simulink model "sschdlexViennaRectifierModel"  (R2026a)
settings: Solver=FixedStepDiscrete  StopTime=0.8  MaxStep=1e-4
PreLoadFcn:
  | % Copyright 2017-2023 The MathWorks, Inc.
  | 
  | %% System Parameters
  | Vs    = 120*sqrt(3); % AC source line-to-line (V, rms)
  | Vpeak = Vs/sqrt(3)*sqrt(2); % AC source line-to-ground (V, peak)
  | R = 0.1;  % Resistance (Ohm)
  | L = 2e-3; % Inductance (H)
  | Vdcnom = 400;  % Nominal output dc voltage (V)
  | Pnom   = 10e3; % Nominal power (W)
  | Imax   = Pnom/(1.5*Vpeak); % Maximum ac current        (A)
  | Inom   = Pnom/Vdcnom;      % Nominal output dc current (A)
  | Iload  = 0.2*Inom;         % Initial load current      (A)
  | 
  | %% Control Parameters
  | fsw = 5e3;        % Switching frequency (Hz)
  | Ts  = 1/(50*fsw); % Fundamental sample time (s)
  | Tsc = 1/(10*fsw); % Control sample time (s)
  | 
  | Kp_vdc = 0.7386; % Proportional gain dc-link voltage controller
  | Ki_vdc = 135.6;  % Integral gain dc-link voltage controller
  | Kp_id  = 8.407;  % Proportional gain d-axis current controller
  | Ki_id  = 1127;   % Integral gain d-axis current controller
  | Kp_iq  = 11.91;  % Proportional gain q-axis current controller
  | Ki_iq  = 3706;   % Integral gain q-axis current controller
  | Kp_vn  = 0.4912; % Proportional gain neutral voltage controller
libraries: ee_lib x27, nesl_utility x13, fl_lib x10, eeTransforms x4, slpidlib x4, eeGeneralControl x4, eePwmGeneratorViennaRectifier x1, eeSinusoidalMeasurement x1, eePowerMeasurement x1
(part 2 of 2)

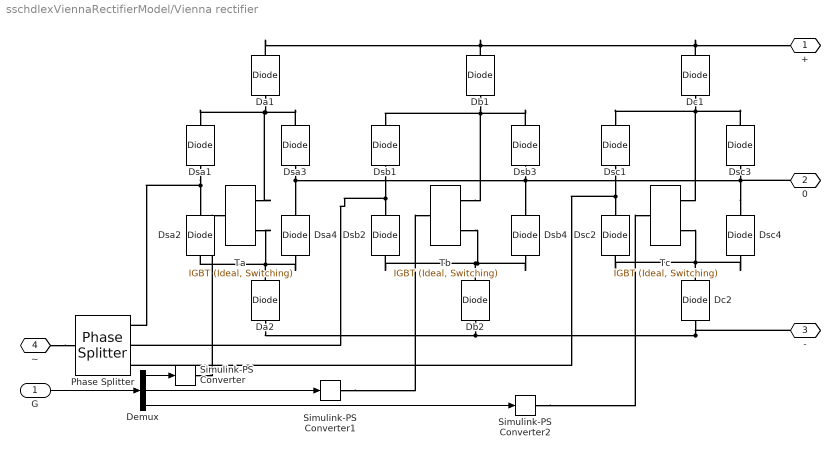
== system sschdlexViennaRectifierModel/Vienna rectifier ==
  G : Inport
  Da1 : ee_lib/Semiconductors & Converters/Diode  ModelType=ee.enum.diode.modelType.pwl  TableType=ee.enum.diode.tableType.IfMat  IfMat=[.07, .12, .19, 1.75, 4.24, 7.32, 11.2; .16, .3, .72, 2.14, 4.02, 6.35, 9.12] A  VfMat=[.9, 1.15, 1.25, 1.5, 1.75, 2.17, 2.6, 2.85; .58, .68, .75, 1.1, 1.38, 1.77, 2.27, 2.7] V  TjVec=[25, 125] degC  VfVec=[.5, .7, .9, 1.3, 1.7, 2.1, 2.5] V  IfVec=[.1, .2, .5, 1, 2, 4, 7, 10] A  IrMat=[1e-06, 2e-06, 5e-06, 1e-05, 2.5e-05, 5e-05, .0001; 2e-06, 5e-06, 1e-05, 4e-05, 8e-05, .0002, .0005] A  VrMat=[10, 100, 200, 250, 300, 325, 350; 10, 70, 160, 220, 270, 300, 320] V  VrVec=[10, 20, 40, 50, 70, 80, 100] V  IrVec=[1e-06, 2e-06, 5e-06, 1e-05, 2e-05, 5e-05, .0001] A  Vf=0.8 V  Ron=0.001 Ohm  Goff=1e-5 1/Ohm  prmExp=ee.enum.diode.expParam.useTwo  I12=[.0137, .545] A  V12=[.6, .7] V  RS=0 Ohm  Tmeas=25 degC  IS=1e-12 A  ec=1  I1=0.0137 A  V1=0.6 V  N_series=1  N_parallel=1  ZenerEnable=false  Rz=0.3 Ohm  BV=inf V  C_param=ee.enum.diode.capParam.fixed  CJ=0 pF  CJ0=5 pF  Vvec=[.1, 10, 100] V  Cvec=[3.5, 1, .4] pF  VJ=1 V  Mgrad=0.5  FC=0.5  Q_param=ee.enum.diode.recoveryParam.off  iRM=-7.15 A  iF=4 A  didt=-750 A/us  trr_factor=3  trr=115 ns  Qrr=1500 s*uA  Vr=-600 V  Ls=150 nH  Erec=0.03 J  TT=50 ns  tau=100 ns  T_param=ee.enum.diode.temperatureParam.off  Tdevice=25 degC  I1_T2=0.245 A  V1_T2=0.5 V  IS_T2=1.25e-7 A  Tmeas2=125 degC  XTI_param=ee.enum.diode.xtiParam.pn  XTI=3  EG_param=ee.enum.diode.egapParam.material_si  EG=1.11 eV  dBVdT=0 V/K  enable_fault_input=simscape.enum.onoff.off  i_specify=off  i_priority=None  i=0 A  i_nominal_specify=off  i_nominal_value=1  i_nominal_unit=A  v_specify=off  v_priority=None  v=0 V  v_nominal_specify=off  v_nominal_value=1  v_nominal_unit=V  v_capacitor_specify=off  v_capacitor_priority=None  v_capacitor=0 V  v_capacitor_nominal_specify=off  v_capacitor_nominal_value=1  v_capacitor_nominal_unit=V  Qj_specify=off  Qj_priority=High  Qj=0 C  Qj_nominal_specify=off  Qj_nominal_value=1  Qj_nominal_unit=C  i_diode_specify=off  i_diode_priority=None  i_diode=0 A  i_diode_nominal_specify=off  i_diode_nominal_value=1  i_diode_nominal_unit=A  v_diode_specify=off  v_diode_priority=None  v_diode=0 V  v_diode_nominal_specify=off  v_diode_nominal_value=1  v_diode_nominal_unit=V  i_capacitor_specify=off  i_capacitor_priority=None  i_capacitor=0 A  i_capacitor_nominal_specify=off  i_capacitor_nominal_value=1  i_capacitor_nominal_unit=A  fidelity_level=ee.enum.diode.fidelity.includeChargeDyn  rec_loss_model=ee.enum.diode.reverseRecoveryModel.fixed  ErecVal=0 J  scaleWithIandV=true  ErecMat=zeros(2, 3) J  ErecMat3D=zeros(2, 3, 2) J  TjrecVec=[298.15, 398.15] K  IfrecVec=[.1, 1, 10] A  IrecVal=10 A  VrecVal=10 V  VrecVec=[0, 100] V  tFilter=1 / 1000 / 100 s  thermal_network_parameterization=ee.enum.thermalNetworkTopology.junctionCase  Rth=[0, 10] K/W  Rth_Cauer=[1, 3, 10] K/W  Rth_Foster=[4, 6] K/W  thermal_mass_parameterization=ee.enum.thermalNetwork.timeconstant  thermal_mass=[0, 1] J/K  thermal_mass_Cauer=[.1, .3, 1] J/K  thermal_mass_Foster=[1.5, 3] J/K  thermal_time_constant=[0, 10] s  thermal_time_constant_Cauer=[1, 3, 10] s  thermal_time_constant_Foster=[6, 18] s  thermal_mass_initial_temperatures=[25, 25] degC  thermal_mass_initial_temperatures_Cauer=[25, 25, 25] degC  junction_thermal_mass=0.01 J/K  Tvec_initial_Foster=[25, 25, 25, 25] degC  no_thermal_network=0  junction_temperature_specify=off  junction_temperature_priority=None  junction_temperature=25 degC  junction_temperature_nominal_specify=off  junction_temperature_nominal_value=1  junction_temperature_nominal_unit=degC
  Da2 : ee_lib/Semiconductors & Converters/Diode  ModelType=ee.enum.diode.modelType.pwl  TableType=ee.enum.diode.tableType.IfMat  IfMat=[.07, .12, .19, 1.75, 4.24, 7.32, 11.2; .16, .3, .72, 2.14, 4.02, 6.35, 9.12] A  VfMat=[.9, 1.15, 1.25, 1.5, 1.75, 2.17, 2.6, 2.85; .58, .68, .75, 1.1, 1.38, 1.77, 2.27, 2.7] V  TjVec=[25, 125] degC  VfVec=[.5, .7, .9, 1.3, 1.7, 2.1, 2.5] V  IfVec=[.1, .2, .5, 1, 2, 4, 7, 10] A  IrMat=[1e-06, 2e-06, 5e-06, 1e-05, 2.5e-05, 5e-05, .0001; 2e-06, 5e-06, 1e-05, 4e-05, 8e-05, .0002, .0005] A  VrMat=[10, 100, 200, 250, 300, 325, 350; 10, 70, 160, 220, 270, 300, 320] V  VrVec=[10, 20, 40, 50, 70, 80, 100] V  IrVec=[1e-06, 2e-06, 5e-06, 1e-05, 2e-05, 5e-05, .0001] A  Vf=0.8 V  Ron=0.001 Ohm  Goff=1e-5 1/Ohm  prmExp=ee.enum.diode.expParam.useTwo  I12=[.0137, .545] A  V12=[.6, .7] V  RS=0 Ohm  Tmeas=25 degC  IS=1e-12 A  ec=1  I1=0.0137 A  V1=0.6 V  N_series=1  N_parallel=1  ZenerEnable=false  Rz=0.3 Ohm  BV=inf V  C_param=ee.enum.diode.capParam.fixed  CJ=0 pF  CJ0=5 pF  Vvec=[.1, 10, 100] V  Cvec=[3.5, 1, .4] pF  VJ=1 V  Mgrad=0.5  FC=0.5  Q_param=ee.enum.diode.recoveryParam.off  iRM=-7.15 A  iF=4 A  didt=-750 A/us  trr_factor=3  trr=115 ns  Qrr=1500 s*uA  Vr=-600 V  Ls=150 nH  Erec=0.03 J  TT=50 ns  tau=100 ns  T_param=ee.enum.diode.temperatureParam.off  Tdevice=25 degC  I1_T2=0.245 A  V1_T2=0.5 V  IS_T2=1.25e-7 A  Tmeas2=125 degC  XTI_param=ee.enum.diode.xtiParam.pn  XTI=3  EG_param=ee.enum.diode.egapParam.material_si  EG=1.11 eV  dBVdT=0 V/K  enable_fault_input=simscape.enum.onoff.off  i_specify=off  i_priority=None  i=0 A  i_nominal_specify=off  i_nominal_value=1  i_nominal_unit=A  v_specify=off  v_priority=None  v=0 V  v_nominal_specify=off  v_nominal_value=1  v_nominal_unit=V  v_capacitor_specify=off  v_capacitor_priority=None  v_capacitor=0 V  v_capacitor_nominal_specify=off  v_capacitor_nominal_value=1  v_capacitor_nominal_unit=V  Qj_specify=off  Qj_priority=High  Qj=0 C  Qj_nominal_specify=off  Qj_nominal_value=1  Qj_nominal_unit=C  i_diode_specify=off  i_diode_priority=None  i_diode=0 A  i_diode_nominal_specify=off  i_diode_nominal_value=1  i_diode_nominal_unit=A  v_diode_specify=off  v_diode_priority=None  v_diode=0 V  v_diode_nominal_specify=off  v_diode_nominal_value=1  v_diode_nominal_unit=V  i_capacitor_specify=off  i_capacitor_priority=None  i_capacitor=0 A  i_capacitor_nominal_specify=off  i_capacitor_nominal_value=1  i_capacitor_nominal_unit=A  fidelity_level=ee.enum.diode.fidelity.includeChargeDyn  rec_loss_model=ee.enum.diode.reverseRecoveryModel.fixed  ErecVal=0 J  scaleWithIandV=true  ErecMat=zeros(2, 3) J  ErecMat3D=zeros(2, 3, 2) J  TjrecVec=[298.15, 398.15] K  IfrecVec=[.1, 1, 10] A  IrecVal=10 A  VrecVal=10 V  VrecVec=[0, 100] V  tFilter=1 / 1000 / 100 s  thermal_network_parameterization=ee.enum.thermalNetworkTopology.junctionCase  Rth=[0, 10] K/W  Rth_Cauer=[1, 3, 10] K/W  Rth_Foster=[4, 6] K/W  thermal_mass_parameterization=ee.enum.thermalNetwork.timeconstant  thermal_mass=[0, 1] J/K  thermal_mass_Cauer=[.1, .3, 1] J/K  thermal_mass_Foster=[1.5, 3] J/K  thermal_time_constant=[0, 10] s  thermal_time_constant_Cauer=[1, 3, 10] s  thermal_time_constant_Foster=[6, 18] s  thermal_mass_initial_temperatures=[25, 25] degC  thermal_mass_initial_temperatures_Cauer=[25, 25, 25] degC  junction_thermal_mass=0.01 J/K  Tvec_initial_Foster=[25, 25, 25, 25] degC  no_thermal_network=0  junction_temperature_specify=off  junction_temperature_priority=None  junction_temperature=25 degC  junction_temperature_nominal_specify=off  junction_temperature_nominal_value=1  junction_temperature_nominal_unit=degC
  Db1 : ee_lib/Semiconductors & Converters/Diode  ModelType=ee.enum.diode.modelType.pwl  TableType=ee.enum.diode.tableType.IfMat  IfMat=[.07, .12, .19, 1.75, 4.24, 7.32, 11.2; .16, .3, .72, 2.14, 4.02, 6.35, 9.12] A  VfMat=[.9, 1.15, 1.25, 1.5, 1.75, 2.17, 2.6, 2.85; .58, .68, .75, 1.1, 1.38, 1.77, 2.27, 2.7] V  TjVec=[25, 125] degC  VfVec=[.5, .7, .9, 1.3, 1.7, 2.1, 2.5] V  IfVec=[.1, .2, .5, 1, 2, 4, 7, 10] A  IrMat=[1e-06, 2e-06, 5e-06, 1e-05, 2.5e-05, 5e-05, .0001; 2e-06, 5e-06, 1e-05, 4e-05, 8e-05, .0002, .0005] A  VrMat=[10, 100, 200, 250, 300, 325, 350; 10, 70, 160, 220, 270, 300, 320] V  VrVec=[10, 20, 40, 50, 70, 80, 100] V  IrVec=[1e-06, 2e-06, 5e-06, 1e-05, 2e-05, 5e-05, .0001] A  Vf=0.8 V  Ron=0.001 Ohm  Goff=1e-5 1/Ohm  prmExp=ee.enum.diode.expParam.useTwo  I12=[.0137, .545] A  V12=[.6, .7] V  RS=0 Ohm  Tmeas=25 degC  IS=1e-12 A  ec=1  I1=0.0137 A  V1=0.6 V  N_series=1  N_parallel=1  ZenerEnable=false  Rz=0.3 Ohm  BV=inf V  C_param=ee.enum.diode.capParam.fixed  CJ=0 pF  CJ0=5 pF  Vvec=[.1, 10, 100] V  Cvec=[3.5, 1, .4] pF  VJ=1 V  Mgrad=0.5  FC=0.5  Q_param=ee.enum.diode.recoveryParam.off  iRM=-7.15 A  iF=4 A  didt=-750 A/us  trr_factor=3  trr=115 ns  Qrr=1500 s*uA  Vr=-600 V  Ls=150 nH  Erec=0.03 J  TT=50 ns  tau=100 ns  T_param=ee.enum.diode.temperatureParam.off  Tdevice=25 degC  I1_T2=0.245 A  V1_T2=0.5 V  IS_T2=1.25e-7 A  Tmeas2=125 degC  XTI_param=ee.enum.diode.xtiParam.pn  XTI=3  EG_param=ee.enum.diode.egapParam.material_si  EG=1.11 eV  dBVdT=0 V/K  enable_fault_input=simscape.enum.onoff.off  i_specify=off  i_priority=None  i=0 A  i_nominal_specify=off  i_nominal_value=1  i_nominal_unit=A  v_specify=off  v_priority=None  v=0 V  v_nominal_specify=off  v_nominal_value=1  v_nominal_unit=V  v_capacitor_specify=off  v_capacitor_priority=None  v_capacitor=0 V  v_capacitor_nominal_specify=off  v_capacitor_nominal_value=1  v_capacitor_nominal_unit=V  Qj_specify=off  Qj_priority=High  Qj=0 C  Qj_nominal_specify=off  Qj_nominal_value=1  Qj_nominal_unit=C  i_diode_specify=off  i_diode_priority=None  i_diode=0 A  i_diode_nominal_specify=off  i_diode_nominal_value=1  i_diode_nominal_unit=A  v_diode_specify=off  v_diode_priority=None  v_diode=0 V  v_diode_nominal_specify=off  v_diode_nominal_value=1  v_diode_nominal_unit=V  i_capacitor_specify=off  i_capacitor_priority=None  i_capacitor=0 A  i_capacitor_nominal_specify=off  i_capacitor_nominal_value=1  i_capacitor_nominal_unit=A  fidelity_level=ee.enum.diode.fidelity.includeChargeDyn  rec_loss_model=ee.enum.diode.reverseRecoveryModel.fixed  ErecVal=0 J  scaleWithIandV=true  ErecMat=zeros(2, 3) J  ErecMat3D=zeros(2, 3, 2) J  TjrecVec=[298.15, 398.15] K  IfrecVec=[.1, 1, 10] A  IrecVal=10 A  VrecVal=10 V  VrecVec=[0, 100] V  tFilter=1 / 1000 / 100 s  thermal_network_parameterization=ee.enum.thermalNetworkTopology.junctionCase  Rth=[0, 10] K/W  Rth_Cauer=[1, 3, 10] K/W  Rth_Foster=[4, 6] K/W  thermal_mass_parameterization=ee.enum.thermalNetwork.timeconstant  thermal_mass=[0, 1] J/K  thermal_mass_Cauer=[.1, .3, 1] J/K  thermal_mass_Foster=[1.5, 3] J/K  thermal_time_constant=[0, 10] s  thermal_time_constant_Cauer=[1, 3, 10] s  thermal_time_constant_Foster=[6, 18] s  thermal_mass_initial_temperatures=[25, 25] degC  thermal_mass_initial_temperatures_Cauer=[25, 25, 25] degC  junction_thermal_mass=0.01 J/K  Tvec_initial_Foster=[25, 25, 25, 25] degC  no_thermal_network=0  junction_temperature_specify=off  junction_temperature_priority=None  junction_temperature=25 degC  junction_temperature_nominal_specify=off  junction_temperature_nominal_value=1  junction_temperature_nominal_unit=degC
  Db2 : ee_lib/Semiconductors & Converters/Diode  ModelType=ee.enum.diode.modelType.pwl  TableType=ee.enum.diode.tableType.IfMat  IfMat=[.07, .12, .19, 1.75, 4.24, 7.32, 11.2; .16, .3, .72, 2.14, 4.02, 6.35, 9.12] A  VfMat=[.9, 1.15, 1.25, 1.5, 1.75, 2.17, 2.6, 2.85; .58, .68, .75, 1.1, 1.38, 1.77, 2.27, 2.7] V  TjVec=[25, 125] degC  VfVec=[.5, .7, .9, 1.3, 1.7, 2.1, 2.5] V  IfVec=[.1, .2, .5, 1, 2, 4, 7, 10] A  IrMat=[1e-06, 2e-06, 5e-06, 1e-05, 2.5e-05, 5e-05, .0001; 2e-06, 5e-06, 1e-05, 4e-05, 8e-05, .0002, .0005] A  VrMat=[10, 100, 200, 250, 300, 325, 350; 10, 70, 160, 220, 270, 300, 320] V  VrVec=[10, 20, 40, 50, 70, 80, 100] V  IrVec=[1e-06, 2e-06, 5e-06, 1e-05, 2e-05, 5e-05, .0001] A  Vf=0.8 V  Ron=0.001 Ohm  Goff=1e-5 1/Ohm  prmExp=ee.enum.diode.expParam.useTwo  I12=[.0137, .545] A  V12=[.6, .7] V  RS=0 Ohm  Tmeas=25 degC  IS=1e-12 A  ec=1  I1=0.0137 A  V1=0.6 V  N_series=1  N_parallel=1  ZenerEnable=false  Rz=0.3 Ohm  BV=inf V  C_param=ee.enum.diode.capParam.fixed  CJ=0 pF  CJ0=5 pF  Vvec=[.1, 10, 100] V  Cvec=[3.5, 1, .4] pF  VJ=1 V  Mgrad=0.5  FC=0.5  Q_param=ee.enum.diode.recoveryParam.off  iRM=-7.15 A  iF=4 A  didt=-750 A/us  trr_factor=3  trr=115 ns  Qrr=1500 s*uA  Vr=-600 V  Ls=150 nH  Erec=0.03 J  TT=50 ns  tau=100 ns  T_param=ee.enum.diode.temperatureParam.off  Tdevice=25 degC  I1_T2=0.245 A  V1_T2=0.5 V  IS_T2=1.25e-7 A  Tmeas2=125 degC  XTI_param=ee.enum.diode.xtiParam.pn  XTI=3  EG_param=ee.enum.diode.egapParam.material_si  EG=1.11 eV  dBVdT=0 V/K  enable_fault_input=simscape.enum.onoff.off  i_specify=off  i_priority=None  i=0 A  i_nominal_specify=off  i_nominal_value=1  i_nominal_unit=A  v_specify=off  v_priority=None  v=0 V  v_nominal_specify=off  v_nominal_value=1  v_nominal_unit=V  v_capacitor_specify=off  v_capacitor_priority=None  v_capacitor=0 V  v_capacitor_nominal_specify=off  v_capacitor_nominal_value=1  v_capacitor_nominal_unit=V  Qj_specify=off  Qj_priority=High  Qj=0 C  Qj_nominal_specify=off  Qj_nominal_value=1  Qj_nominal_unit=C  i_diode_specify=off  i_diode_priority=None  i_diode=0 A  i_diode_nominal_specify=off  i_diode_nominal_value=1  i_diode_nominal_unit=A  v_diode_specify=off  v_diode_priority=None  v_diode=0 V  v_diode_nominal_specify=off  v_diode_nominal_value=1  v_diode_nominal_unit=V  i_capacitor_specify=off  i_capacitor_priority=None  i_capacitor=0 A  i_capacitor_nominal_specify=off  i_capacitor_nominal_value=1  i_capacitor_nominal_unit=A  fidelity_level=ee.enum.diode.fidelity.includeChargeDyn  rec_loss_model=ee.enum.diode.reverseRecoveryModel.fixed  ErecVal=0 J  scaleWithIandV=true  ErecMat=zeros(2, 3) J  ErecMat3D=zeros(2, 3, 2) J  TjrecVec=[298.15, 398.15] K  IfrecVec=[.1, 1, 10] A  IrecVal=10 A  VrecVal=10 V  VrecVec=[0, 100] V  tFilter=1 / 1000 / 100 s  thermal_network_parameterization=ee.enum.thermalNetworkTopology.junctionCase  Rth=[0, 10] K/W  Rth_Cauer=[1, 3, 10] K/W  Rth_Foster=[4, 6] K/W  thermal_mass_parameterization=ee.enum.thermalNetwork.timeconstant  thermal_mass=[0, 1] J/K  thermal_mass_Cauer=[.1, .3, 1] J/K  thermal_mass_Foster=[1.5, 3] J/K  thermal_time_constant=[0, 10] s  thermal_time_constant_Cauer=[1, 3, 10] s  thermal_time_constant_Foster=[6, 18] s  thermal_mass_initial_temperatures=[25, 25] degC  thermal_mass_initial_temperatures_Cauer=[25, 25, 25] degC  junction_thermal_mass=0.01 J/K  Tvec_initial_Foster=[25, 25, 25, 25] degC  no_thermal_network=0  junction_temperature_specify=off  junction_temperature_priority=None  junction_temperature=25 degC  junction_temperature_nominal_specify=off  junction_temperature_nominal_value=1  junction_temperature_nominal_unit=degC
  Dc1 : ee_lib/Semiconductors & Converters/Diode  ModelType=ee.enum.diode.modelType.pwl  TableType=ee.enum.diode.tableType.IfMat  IfMat=[.07, .12, .19, 1.75, 4.24, 7.32, 11.2; .16, .3, .72, 2.14, 4.02, 6.35, 9.12] A  VfMat=[.9, 1.15, 1.25, 1.5, 1.75, 2.17, 2.6, 2.85; .58, .68, .75, 1.1, 1.38, 1.77, 2.27, 2.7] V  TjVec=[25, 125] degC  VfVec=[.5, .7, .9, 1.3, 1.7, 2.1, 2.5] V  IfVec=[.1, .2, .5, 1, 2, 4, 7, 10] A  IrMat=[1e-06, 2e-06, 5e-06, 1e-05, 2.5e-05, 5e-05, .0001; 2e-06, 5e-06, 1e-05, 4e-05, 8e-05, .0002, .0005] A  VrMat=[10, 100, 200, 250, 300, 325, 350; 10, 70, 160, 220, 270, 300, 320] V  VrVec=[10, 20, 40, 50, 70, 80, 100] V  IrVec=[1e-06, 2e-06, 5e-06, 1e-05, 2e-05, 5e-05, .0001] A  Vf=0.8 V  Ron=0.001 Ohm  Goff=1e-5 1/Ohm  prmExp=ee.enum.diode.expParam.useTwo  I12=[.0137, .545] A  V12=[.6, .7] V  RS=0 Ohm  Tmeas=25 degC  IS=1e-12 A  ec=1  I1=0.0137 A  V1=0.6 V  N_series=1  N_parallel=1  ZenerEnable=false  Rz=0.3 Ohm  BV=inf V  C_param=ee.enum.diode.capParam.fixed  CJ=0 pF  CJ0=5 pF  Vvec=[.1, 10, 100] V  Cvec=[3.5, 1, .4] pF  VJ=1 V  Mgrad=0.5  FC=0.5  Q_param=ee.enum.diode.recoveryParam.off  iRM=-7.15 A  iF=4 A  didt=-750 A/us  trr_factor=3  trr=115 ns  Qrr=1500 s*uA  Vr=-600 V  Ls=150 nH  Erec=0.03 J  TT=50 ns  tau=100 ns  T_param=ee.enum.diode.temperatureParam.off  Tdevice=25 degC  I1_T2=0.245 A  V1_T2=0.5 V  IS_T2=1.25e-7 A  Tmeas2=125 degC  XTI_param=ee.enum.diode.xtiParam.pn  XTI=3  EG_param=ee.enum.diode.egapParam.material_si  EG=1.11 eV  dBVdT=0 V/K  enable_fault_input=simscape.enum.onoff.off  i_specify=off  i_priority=None  i=0 A  i_nominal_specify=off  i_nominal_value=1  i_nominal_unit=A  v_specify=off  v_priority=None  v=0 V  v_nominal_specify=off  v_nominal_value=1  v_nominal_unit=V  v_capacitor_specify=off  v_capacitor_priority=None  v_capacitor=0 V  v_capacitor_nominal_specify=off  v_capacitor_nominal_value=1  v_capacitor_nominal_unit=V  Qj_specify=off  Qj_priority=High  Qj=0 C  Qj_nominal_specify=off  Qj_nominal_value=1  Qj_nominal_unit=C  i_diode_specify=off  i_diode_priority=None  i_diode=0 A  i_diode_nominal_specify=off  i_diode_nominal_value=1  i_diode_nominal_unit=A  v_diode_specify=off  v_diode_priority=None  v_diode=0 V  v_diode_nominal_specify=off  v_diode_nominal_value=1  v_diode_nominal_unit=V  i_capacitor_specify=off  i_capacitor_priority=None  i_capacitor=0 A  i_capacitor_nominal_specify=off  i_capacitor_nominal_value=1  i_capacitor_nominal_unit=A  fidelity_level=ee.enum.diode.fidelity.includeChargeDyn  rec_loss_model=ee.enum.diode.reverseRecoveryModel.fixed  ErecVal=0 J  scaleWithIandV=true  ErecMat=zeros(2, 3) J  ErecMat3D=zeros(2, 3, 2) J  TjrecVec=[298.15, 398.15] K  IfrecVec=[.1, 1, 10] A  IrecVal=10 A  VrecVal=10 V  VrecVec=[0, 100] V  tFilter=1 / 1000 / 100 s  thermal_network_parameterization=ee.enum.thermalNetworkTopology.junctionCase  Rth=[0, 10] K/W  Rth_Cauer=[1, 3, 10] K/W  Rth_Foster=[4, 6] K/W  thermal_mass_parameterization=ee.enum.thermalNetwork.timeconstant  thermal_mass=[0, 1] J/K  thermal_mass_Cauer=[.1, .3, 1] J/K  thermal_mass_Foster=[1.5, 3] J/K  thermal_time_constant=[0, 10] s  thermal_time_constant_Cauer=[1, 3, 10] s  thermal_time_constant_Foster=[6, 18] s  thermal_mass_initial_temperatures=[25, 25] degC  thermal_mass_initial_temperatures_Cauer=[25, 25, 25] degC  junction_thermal_mass=0.01 J/K  Tvec_initial_Foster=[25, 25, 25, 25] degC  no_thermal_network=0  junction_temperature_specify=off  junction_temperature_priority=None  junction_temperature=25 degC  junction_temperature_nominal_specify=off  junction_temperature_nominal_value=1  junction_temperature_nominal_unit=degC
  Dc2 : ee_lib/Semiconductors & Converters/Diode  ModelType=ee.enum.diode.modelType.pwl  TableType=ee.enum.diode.tableType.IfMat  IfMat=[.07, .12, .19, 1.75, 4.24, 7.32, 11.2; .16, .3, .72, 2.14, 4.02, 6.35, 9.12] A  VfMat=[.9, 1.15, 1.25, 1.5, 1.75, 2.17, 2.6, 2.85; .58, .68, .75, 1.1, 1.38, 1.77, 2.27, 2.7] V  TjVec=[25, 125] degC  VfVec=[.5, .7, .9, 1.3, 1.7, 2.1, 2.5] V  IfVec=[.1, .2, .5, 1, 2, 4, 7, 10] A  IrMat=[1e-06, 2e-06, 5e-06, 1e-05, 2.5e-05, 5e-05, .0001; 2e-06, 5e-06, 1e-05, 4e-05, 8e-05, .0002, .0005] A  VrMat=[10, 100, 200, 250, 300, 325, 350; 10, 70, 160, 220, 270, 300, 320] V  VrVec=[10, 20, 40, 50, 70, 80, 100] V  IrVec=[1e-06, 2e-06, 5e-06, 1e-05, 2e-05, 5e-05, .0001] A  Vf=0.8 V  Ron=0.001 Ohm  Goff=1e-5 1/Ohm  prmExp=ee.enum.diode.expParam.useTwo  I12=[.0137, .545] A  V12=[.6, .7] V  RS=0 Ohm  Tmeas=25 degC  IS=1e-12 A  ec=1  I1=0.0137 A  V1=0.6 V  N_series=1  N_parallel=1  ZenerEnable=false  Rz=0.3 Ohm  BV=inf V  C_param=ee.enum.diode.capParam.fixed  CJ=0 pF  CJ0=5 pF  Vvec=[.1, 10, 100] V  Cvec=[3.5, 1, .4] pF  VJ=1 V  Mgrad=0.5  FC=0.5  Q_param=ee.enum.diode.recoveryParam.off  iRM=-7.15 A  iF=4 A  didt=-750 A/us  trr_factor=3  trr=115 ns  Qrr=1500 s*uA  Vr=-600 V  Ls=150 nH  Erec=0.03 J  TT=50 ns  tau=100 ns  T_param=ee.enum.diode.temperatureParam.off  Tdevice=25 degC  I1_T2=0.245 A  V1_T2=0.5 V  IS_T2=1.25e-7 A  Tmeas2=125 degC  XTI_param=ee.enum.diode.xtiParam.pn  XTI=3  EG_param=ee.enum.diode.egapParam.material_si  EG=1.11 eV  dBVdT=0 V/K  enable_fault_input=simscape.enum.onoff.off  i_specify=off  i_priority=None  i=0 A  i_nominal_specify=off  i_nominal_value=1  i_nominal_unit=A  v_specify=off  v_priority=None  v=0 V  v_nominal_specify=off  v_nominal_value=1  v_nominal_unit=V  v_capacitor_specify=off  v_capacitor_priority=None  v_capacitor=0 V  v_capacitor_nominal_specify=off  v_capacitor_nominal_value=1  v_capacitor_nominal_unit=V  Qj_specify=off  Qj_priority=High  Qj=0 C  Qj_nominal_specify=off  Qj_nominal_value=1  Qj_nominal_unit=C  i_diode_specify=off  i_diode_priority=None  i_diode=0 A  i_diode_nominal_specify=off  i_diode_nominal_value=1  i_diode_nominal_unit=A  v_diode_specify=off  v_diode_priority=None  v_diode=0 V  v_diode_nominal_specify=off  v_diode_nominal_value=1  v_diode_nominal_unit=V  i_capacitor_specify=off  i_capacitor_priority=None  i_capacitor=0 A  i_capacitor_nominal_specify=off  i_capacitor_nominal_value=1  i_capacitor_nominal_unit=A  fidelity_level=ee.enum.diode.fidelity.includeChargeDyn  rec_loss_model=ee.enum.diode.reverseRecoveryModel.fixed  ErecVal=0 J  scaleWithIandV=true  ErecMat=zeros(2, 3) J  ErecMat3D=zeros(2, 3, 2) J  TjrecVec=[298.15, 398.15] K  IfrecVec=[.1, 1, 10] A  IrecVal=10 A  VrecVal=10 V  VrecVec=[0, 100] V  tFilter=1 / 1000 / 100 s  thermal_network_parameterization=ee.enum.thermalNetworkTopology.junctionCase  Rth=[0, 10] K/W  Rth_Cauer=[1, 3, 10] K/W  Rth_Foster=[4, 6] K/W  thermal_mass_parameterization=ee.enum.thermalNetwork.timeconstant  thermal_mass=[0, 1] J/K  thermal_mass_Cauer=[.1, .3, 1] J/K  thermal_mass_Foster=[1.5, 3] J/K  thermal_time_constant=[0, 10] s  thermal_time_constant_Cauer=[1, 3, 10] s  thermal_time_constant_Foster=[6, 18] s  thermal_mass_initial_temperatures=[25, 25] degC  thermal_mass_initial_temperatures_Cauer=[25, 25, 25] degC  junction_thermal_mass=0.01 J/K  Tvec_initial_Foster=[25, 25, 25, 25] degC  no_thermal_network=0  junction_temperature_specify=off  junction_temperature_priority=None  junction_temperature=25 degC  junction_temperature_nominal_specify=off  junction_temperature_nominal_value=1  junction_temperature_nominal_unit=degC
  Demux : Demux  Outputs=3
  Dsa{1..4} (4 alike) : ee_lib/Semiconductors & Converters/Diode  ModelType=ee.enum.diode.modelType.pwl  TableType=ee.enum.diode.tableType.IfMat  IfMat=[.07, .12, .19, 1.75, 4.24, 7.32, 11.2; .16, .3, .72, 2.14, 4.02, 6.35, 9.12] A  VfMat=[.9, 1.15, 1.25, 1.5, 1.75, 2.17, 2.6, 2.85; .58, .68, .75, 1.1, 1.38, 1.77, 2.27, 2.7] V  TjVec=[25, 125] degC  VfVec=[.5, .7, .9, 1.3, 1.7, 2.1, 2.5] V  IfVec=[.1, .2, .5, 1, 2, 4, 7, 10] A  IrMat=[1e-06, 2e-06, 5e-06, 1e-05, 2.5e-05, 5e-05, .0001; 2e-06, 5e-06, 1e-05, 4e-05, 8e-05, .0002, .0005] A  VrMat=[10, 100, 200, 250, 300, 325, 350; 10, 70, 160, 220, 270, 300, 320] V  VrVec=[10, 20, 40, 50, 70, 80, 100] V  IrVec=[1e-06, 2e-06, 5e-06, 1e-05, 2e-05, 5e-05, .0001] A  Vf=0.8 V  Ron=0.001 Ohm  Goff=1e-5 1/Ohm  prmExp=ee.enum.diode.expParam.useTwo  I12=[.0137, .545] A  V12=[.6, .7] V  RS=0 Ohm  Tmeas=25 degC  IS=1e-12 A  ec=1  I1=0.0137 A  V1=0.6 V  N_series=1  N_parallel=1  ZenerEnable=false  Rz=0.3 Ohm  BV=inf V  C_param=ee.enum.diode.capParam.fixed  CJ=0 pF  CJ0=5 pF  Vvec=[.1, 10, 100] V  Cvec=[3.5, 1, .4] pF  VJ=1 V  Mgrad=0.5  FC=0.5  Q_param=ee.enum.diode.recoveryParam.off  iRM=-7.15 A  iF=4 A  didt=-750 A/us  trr_factor=3  trr=115 ns  Qrr=1500 s*uA  Vr=-600 V  Ls=150 nH  Erec=0.03 J  TT=50 ns  tau=100 ns  T_param=ee.enum.diode.temperatureParam.off  Tdevice=25 degC  I1_T2=0.245 A  V1_T2=0.5 V  IS_T2=1.25e-7 A  Tmeas2=125 degC  XTI_param=ee.enum.diode.xtiParam.pn  XTI=3  EG_param=ee.enum.diode.egapParam.material_si  EG=1.11 eV  dBVdT=0 V/K  enable_fault_input=simscape.enum.onoff.off  i_specify=off  i_priority=None  i=0 A  i_nominal_specify=off  i_nominal_value=1  i_nominal_unit=A  v_specify=off  v_priority=None  v=0 V  v_nominal_specify=off  v_nominal_value=1  v_nominal_unit=V  v_capacitor_specify=off  v_capacitor_priority=None  v_capacitor=0 V  v_capacitor_nominal_specify=off  v_capacitor_nominal_value=1  v_capacitor_nominal_unit=V  Qj_specify=off  Qj_priority=High  Qj=0 C  Qj_nominal_specify=off  Qj_nominal_value=1  Qj_nominal_unit=C  i_diode_specify=off  i_diode_priority=None  i_diode=0 A  i_diode_nominal_specify=off  i_diode_nominal_value=1  i_diode_nominal_unit=A  v_diode_specify=off  v_diode_priority=None  v_diode=0 V  v_diode_nominal_specify=off  v_diode_nominal_value=1  v_diode_nominal_unit=V  i_capacitor_specify=off  i_capacitor_priority=None  i_capacitor=0 A  i_capacitor_nominal_specify=off  i_capacitor_nominal_value=1  i_capacitor_nominal_unit=A  fidelity_level=ee.enum.diode.fidelity.includeChargeDyn  rec_loss_model=ee.enum.diode.reverseRecoveryModel.fixed  ErecVal=0 J  scaleWithIandV=true  ErecMat=zeros(2, 3) J  ErecMat3D=zeros(2, 3, 2) J  TjrecVec=[298.15, 398.15] K  IfrecVec=[.1, 1, 10] A  IrecVal=10 A  VrecVal=10 V  VrecVec=[0, 100] V  tFilter=1 / 1000 / 100 s  thermal_network_parameterization=ee.enum.thermalNetworkTopology.junctionCase  Rth=[0, 10] K/W  Rth_Cauer=[1, 3, 10] K/W  Rth_Foster=[4, 6] K/W  thermal_mass_parameterization=ee.enum.thermalNetwork.timeconstant  thermal_mass=[0, 1] J/K  thermal_mass_Cauer=[.1, .3, 1] J/K  thermal_mass_Foster=[1.5, 3] J/K  thermal_time_constant=[0, 10] s  thermal_time_constant_Cauer=[1, 3, 10] s  thermal_time_constant_Foster=[6, 18] s  thermal_mass_initial_temperatures=[25, 25] degC  thermal_mass_initial_temperatures_Cauer=[25, 25, 25] degC  junction_thermal_mass=0.01 J/K  Tvec_initial_Foster=[25, 25, 25, 25] degC  no_thermal_network=0  junction_temperature_specify=off  junction_temperature_priority=None  junction_temperature=25 degC  junction_temperature_nominal_specify=off  junction_temperature_nominal_value=1  junction_temperature_nominal_unit=degC
  Dsb{1..4} (4 alike) : ee_lib/Semiconductors & Converters/Diode  ModelType=ee.enum.diode.modelType.pwl  TableType=ee.enum.diode.tableType.IfMat  IfMat=[.07, .12, .19, 1.75, 4.24, 7.32, 11.2; .16, .3, .72, 2.14, 4.02, 6.35, 9.12] A  VfMat=[.9, 1.15, 1.25, 1.5, 1.75, 2.17, 2.6, 2.85; .58, .68, .75, 1.1, 1.38, 1.77, 2.27, 2.7] V  TjVec=[25, 125] degC  VfVec=[.5, .7, .9, 1.3, 1.7, 2.1, 2.5] V  IfVec=[.1, .2, .5, 1, 2, 4, 7, 10] A  IrMat=[1e-06, 2e-06, 5e-06, 1e-05, 2.5e-05, 5e-05, .0001; 2e-06, 5e-06, 1e-05, 4e-05, 8e-05, .0002, .0005] A  VrMat=[10, 100, 200, 250, 300, 325, 350; 10, 70, 160, 220, 270, 300, 320] V  VrVec=[10, 20, 40, 50, 70, 80, 100] V  IrVec=[1e-06, 2e-06, 5e-06, 1e-05, 2e-05, 5e-05, .0001] A  Vf=0.8 V  Ron=0.001 Ohm  Goff=1e-5 1/Ohm  prmExp=ee.enum.diode.expParam.useTwo  I12=[.0137, .545] A  V12=[.6, .7] V  RS=0 Ohm  Tmeas=25 degC  IS=1e-12 A  ec=1  I1=0.0137 A  V1=0.6 V  N_series=1  N_parallel=1  ZenerEnable=false  Rz=0.3 Ohm  BV=inf V  C_param=ee.enum.diode.capParam.fixed  CJ=0 pF  CJ0=5 pF  Vvec=[.1, 10, 100] V  Cvec=[3.5, 1, .4] pF  VJ=1 V  Mgrad=0.5  FC=0.5  Q_param=ee.enum.diode.recoveryParam.off  iRM=-7.15 A  iF=4 A  didt=-750 A/us  trr_factor=3  trr=115 ns  Qrr=1500 s*uA  Vr=-600 V  Ls=150 nH  Erec=0.03 J  TT=50 ns  tau=100 ns  T_param=ee.enum.diode.temperatureParam.off  Tdevice=25 degC  I1_T2=0.245 A  V1_T2=0.5 V  IS_T2=1.25e-7 A  Tmeas2=125 degC  XTI_param=ee.enum.diode.xtiParam.pn  XTI=3  EG_param=ee.enum.diode.egapParam.material_si  EG=1.11 eV  dBVdT=0 V/K  enable_fault_input=simscape.enum.onoff.off  i_specify=off  i_priority=None  i=0 A  i_nominal_specify=off  i_nominal_value=1  i_nominal_unit=A  v_specify=off  v_priority=None  v=0 V  v_nominal_specify=off  v_nominal_value=1  v_nominal_unit=V  v_capacitor_specify=off  v_capacitor_priority=None  v_capacitor=0 V  v_capacitor_nominal_specify=off  v_capacitor_nominal_value=1  v_capacitor_nominal_unit=V  Qj_specify=off  Qj_priority=High  Qj=0 C  Qj_nominal_specify=off  Qj_nominal_value=1  Qj_nominal_unit=C  i_diode_specify=off  i_diode_priority=None  i_diode=0 A  i_diode_nominal_specify=off  i_diode_nominal_value=1  i_diode_nominal_unit=A  v_diode_specify=off  v_diode_priority=None  v_diode=0 V  v_diode_nominal_specify=off  v_diode_nominal_value=1  v_diode_nominal_unit=V  i_capacitor_specify=off  i_capacitor_priority=None  i_capacitor=0 A  i_capacitor_nominal_specify=off  i_capacitor_nominal_value=1  i_capacitor_nominal_unit=A  fidelity_level=ee.enum.diode.fidelity.includeChargeDyn  rec_loss_model=ee.enum.diode.reverseRecoveryModel.fixed  ErecVal=0 J  scaleWithIandV=true  ErecMat=zeros(2, 3) J  ErecMat3D=zeros(2, 3, 2) J  TjrecVec=[298.15, 398.15] K  IfrecVec=[.1, 1, 10] A  IrecVal=10 A  VrecVal=10 V  VrecVec=[0, 100] V  tFilter=1 / 1000 / 100 s  thermal_network_parameterization=ee.enum.thermalNetworkTopology.junctionCase  Rth=[0, 10] K/W  Rth_Cauer=[1, 3, 10] K/W  Rth_Foster=[4, 6] K/W  thermal_mass_parameterization=ee.enum.thermalNetwork.timeconstant  thermal_mass=[0, 1] J/K  thermal_mass_Cauer=[.1, .3, 1] J/K  thermal_mass_Foster=[1.5, 3] J/K  thermal_time_constant=[0, 10] s  thermal_time_constant_Cauer=[1, 3, 10] s  thermal_time_constant_Foster=[6, 18] s  thermal_mass_initial_temperatures=[25, 25] degC  thermal_mass_initial_temperatures_Cauer=[25, 25, 25] degC  junction_thermal_mass=0.01 J/K  Tvec_initial_Foster=[25, 25, 25, 25] degC  no_thermal_network=0  junction_temperature_specify=off  junction_temperature_priority=None  junction_temperature=25 degC  junction_temperature_nominal_specify=off  junction_temperature_nominal_value=1  junction_temperature_nominal_unit=degC
  Dsc{1..4} (4 alike) : ee_lib/Semiconductors & Converters/Diode  ModelType=ee.enum.diode.modelType.pwl  TableType=ee.enum.diode.tableType.IfMat  IfMat=[.07, .12, .19, 1.75, 4.24, 7.32, 11.2; .16, .3, .72, 2.14, 4.02, 6.35, 9.12] A  VfMat=[.9, 1.15, 1.25, 1.5, 1.75, 2.17, 2.6, 2.85; .58, .68, .75, 1.1, 1.38, 1.77, 2.27, 2.7] V  TjVec=[25, 125] degC  VfVec=[.5, .7, .9, 1.3, 1.7, 2.1, 2.5] V  IfVec=[.1, .2, .5, 1, 2, 4, 7, 10] A  IrMat=[1e-06, 2e-06, 5e-06, 1e-05, 2.5e-05, 5e-05, .0001; 2e-06, 5e-06, 1e-05, 4e-05, 8e-05, .0002, .0005] A  VrMat=[10, 100, 200, 250, 300, 325, 350; 10, 70, 160, 220, 270, 300, 320] V  VrVec=[10, 20, 40, 50, 70, 80, 100] V  IrVec=[1e-06, 2e-06, 5e-06, 1e-05, 2e-05, 5e-05, .0001] A  Vf=0.8 V  Ron=0.001 Ohm  Goff=1e-5 1/Ohm  prmExp=ee.enum.diode.expParam.useTwo  I12=[.0137, .545] A  V12=[.6, .7] V  RS=0 Ohm  Tmeas=25 degC  IS=1e-12 A  ec=1  I1=0.0137 A  V1=0.6 V  N_series=1  N_parallel=1  ZenerEnable=false  Rz=0.3 Ohm  BV=inf V  C_param=ee.enum.diode.capParam.fixed  CJ=0 pF  CJ0=5 pF  Vvec=[.1, 10, 100] V  Cvec=[3.5, 1, .4] pF  VJ=1 V  Mgrad=0.5  FC=0.5  Q_param=ee.enum.diode.recoveryParam.off  iRM=-7.15 A  iF=4 A  didt=-750 A/us  trr_factor=3  trr=115 ns  Qrr=1500 s*uA  Vr=-600 V  Ls=150 nH  Erec=0.03 J  TT=50 ns  tau=100 ns  T_param=ee.enum.diode.temperatureParam.off  Tdevice=25 degC  I1_T2=0.245 A  V1_T2=0.5 V  IS_T2=1.25e-7 A  Tmeas2=125 degC  XTI_param=ee.enum.diode.xtiParam.pn  XTI=3  EG_param=ee.enum.diode.egapParam.material_si  EG=1.11 eV  dBVdT=0 V/K  enable_fault_input=simscape.enum.onoff.off  i_specify=off  i_priority=None  i=0 A  i_nominal_specify=off  i_nominal_value=1  i_nominal_unit=A  v_specify=off  v_priority=None  v=0 V  v_nominal_specify=off  v_nominal_value=1  v_nominal_unit=V  v_capacitor_specify=off  v_capacitor_priority=None  v_capacitor=0 V  v_capacitor_nominal_specify=off  v_capacitor_nominal_value=1  v_capacitor_nominal_unit=V  Qj_specify=off  Qj_priority=High  Qj=0 C  Qj_nominal_specify=off  Qj_nominal_value=1  Qj_nominal_unit=C  i_diode_specify=off  i_diode_priority=None  i_diode=0 A  i_diode_nominal_specify=off  i_diode_nominal_value=1  i_diode_nominal_unit=A  v_diode_specify=off  v_diode_priority=None  v_diode=0 V  v_diode_nominal_specify=off  v_diode_nominal_value=1  v_diode_nominal_unit=V  i_capacitor_specify=off  i_capacitor_priority=None  i_capacitor=0 A  i_capacitor_nominal_specify=off  i_capacitor_nominal_value=1  i_capacitor_nominal_unit=A  fidelity_level=ee.enum.diode.fidelity.includeChargeDyn  rec_loss_model=ee.enum.diode.reverseRecoveryModel.fixed  ErecVal=0 J  scaleWithIandV=true  ErecMat=zeros(2, 3) J  ErecMat3D=zeros(2, 3, 2) J  TjrecVec=[298.15, 398.15] K  IfrecVec=[.1, 1, 10] A  IrecVal=10 A  VrecVal=10 V  VrecVec=[0, 100] V  tFilter=1 / 1000 / 100 s  thermal_network_parameterization=ee.enum.thermalNetworkTopology.junctionCase  Rth=[0, 10] K/W  Rth_Cauer=[1, 3, 10] K/W  Rth_Foster=[4, 6] K/W  thermal_mass_parameterization=ee.enum.thermalNetwork.timeconstant  thermal_mass=[0, 1] J/K  thermal_mass_Cauer=[.1, .3, 1] J/K  thermal_mass_Foster=[1.5, 3] J/K  thermal_time_constant=[0, 10] s  thermal_time_constant_Cauer=[1, 3, 10] s  thermal_time_constant_Foster=[6, 18] s  thermal_mass_initial_temperatures=[25, 25] degC  thermal_mass_initial_temperatures_Cauer=[25, 25, 25] degC  junction_thermal_mass=0.01 J/K  Tvec_initial_Foster=[25, 25, 25, 25] degC  no_thermal_network=0  junction_temperature_specify=off  junction_temperature_priority=None  junction_temperature=25 degC  junction_temperature_nominal_specify=off  junction_temperature_nominal_value=1  junction_temperature_nominal_unit=degC
  Phase Splitter : ee_lib/Connectors & References/Phase Splitter
  Simulink-PS Converter : nesl_utility/Simulink-PS Converter  PhysicalDomain=network_engine_domain  SubClassName=ps_input  LeftPortType=input  RightPortType=output  PseudoPeriodic=off  Frequencies=[]  NoiseDistribution=none  NoiseParameters=[]  Unit=1  AffineConversion=off  FilteringAndDerivatives=provide  SimscapeFilterOrder=1  InputFilterTimeConstant=0.001  UdotUserProvided=0
  Simulink-PS Converter1 : nesl_utility/Simulink-PS Converter  PhysicalDomain=network_engine_domain  SubClassName=ps_input  LeftPortType=input  RightPortType=output  PseudoPeriodic=off  Frequencies=[]  NoiseDistribution=none  NoiseParameters=[]  Unit=1  AffineConversion=off  FilteringAndDerivatives=provide  SimscapeFilterOrder=1  InputFilterTimeConstant=0.001  UdotUserProvided=0
  Simulink-PS Converter2 : nesl_utility/Simulink-PS Converter  PhysicalDomain=network_engine_domain  SubClassName=ps_input  LeftPortType=input  RightPortType=output  PseudoPeriodic=off  Frequencies=[]  NoiseDistribution=none  NoiseParameters=[]  Unit=1  AffineConversion=off  FilteringAndDerivatives=provide  SimscapeFilterOrder=1  InputFilterTimeConstant=0.001  UdotUserProvided=0
  Ta : ee_lib/Semiconductors & Converters/IGBT (Ideal, Switching)  port_option=ee.enum.controlport.ps  Vf=0.8 V  Ron=0.001 Ohm  Goff=1e-5 1/Ohm  Vth=0.5 V  diode_param=1  diode_Vf=0.8 V  diode_Ron=0.001 Ohm  diode_Goff=1e-5 1/Ohm  diode_C=5e-8 F  diode_iRM=-235 A  diode_iF=300 A  diode_idot=-50 A/us  diode_trr_param=1  diode_trr_factor=3  diode_trr=15 us  diode_Qrr=1.5e+3 s*uA  ice_specify=off  ice_priority=None  ice=0 A  ice_nominal_specify=off  ice_nominal_value=1  ice_nominal_unit=A  vce_specify=off  vce_priority=None  vce=0 V  vce_nominal_specify=off  vce_nominal_value=1  vce_nominal_unit=V  vge_specify=off  vge_priority=None  vge=0 V  vge_nominal_specify=off  vge_nominal_value=1  vge_nominal_unit=V  thermal_loss_option=ee.enum.converters.thermalLossOption.constantvalues  Von_data=[0, .1, .6, .8, 1, 1.3, 1.6, 2, 2.4; 0, .1, .7, 1, 1.2, 1.5, 1.9, 2.4, 2.8] V  Tj=[298.15, 398.15] K  Iout_data=[0, .1, 1, 5, 10, 20, 40, 70, 100] A  tabulateWithVce=false  Eon_data=[0, .0024, .024, .12, .2, .48, 1.04, 2.16, 3.24; 0, .003, .03, .15, .25, .6, 1.3, 2.7, 4.05] * 1e-3 J  Eoff_data=[0, .0007, .0066, .033, .066, .17, .33, .83, 1.5; 0, .001, .01, .05, .1, .25, .5, 1.2, 2.2] * 1e-3 J  Eon_data_3D=[zeros(2, 9, 3)] J  Eoff_data_3D=[zeros(2, 9, 3)] J  Tj_loss=[298.15, 398.15] K  Iout_data_loss=[0, .1, 1, 5, 10, 20, 40, 70, 100] A  Vce_loss=[0, 150, 300] V  Eon_scalar=22.86e-3 J  Eoff_scalar=17.14e-3 J  Voff=300 V  Iout_scalar=600 A  useCurrentFromPreviousCycle=false  useVoltageFromPreviousCycle=false  diodeModelType=ee.enum.converters.diodeModelType.pwl  diodeTableType=ee.enum.diode.tableType.IfMat  diode_ReverseIVType=ee.enum.diode.diodeReverseIV.constant  diode_IfMat=[.07, .12, .19, 1.75, 4.24, 7.32, 11.2; .16, .3, .72, 2.14, 4.02, 6.35, 9.12] A  diode_VfMat=[.9, 1.15, 1.25, 1.5, 1.75, 2.17, 2.6, 2.85; .58, .68, .75, 1.1, 1.38, 1.77, 2.27, 2.7] V  diode_TjVec=[25, 125] degC  diode_VfVec=[.5, .7, .9, 1.3, 1.7, 2.1, 2.5] V  diode_IfVec=[.1, .2, .5, 1, 2, 4, 7, 10] A  diode_IrMat=[1e-06, 2e-06, 5e-06, 1e-05, 2.5e-05, 5e-05, .0001; 2e-06, 5e-06, 1e-05, 4e-05, 8e-05, .0002, .0005] A  diode_VrMat=[10, 100, 200, 250, 300, 325, 350; 10, 70, 160, 220, 270, 300, 320] V  diode_VrVec=[10, 20, 40, 50, 70, 80, 100] V  diode_IrVec=[1e-06, 2e-06, 5e-06, 1e-05, 2e-05, 5e-05, .0001] A  diode_Vr=-600 V  diode_Ls=150 nH  diode_Erec=0.03 J  diode_rec_loss_model=ee.enum.diode.reverseRecoveryModel.fixed  diode_ErecVal=0 J  diode_scaleWithIandV=true  diode_ErecMat=zeros(2, 3) J  diodeErecMat3D=zeros(2, 3, 2) J  diode_TjrecVec=[298.15, 398.15] K  diode_IfrecVec=[.1, 1, 10] A  diodeVrecVec=[0, 100] V  diode_IrecVal=10 A  diode_VrecVal=10 V  diode_tFilter=1 / 1000 / 100 s  separateThermalPortForDiode=false  thermal_network_parameterization=ee.enum.thermalNetworkTopology.external  Rth=[.08, .5] K/W  Rth_Cauer=[.08, .1, .5] K/W  Rth_Foster=[.08, .14, .22, .16] K/W  thermal_mass_parameterization=ee.enum.thermalNetwork.timeconstant  thermal_mass=[.01, .5] J/K  thermal_mass_Cauer=[.01, .1, .5] J/K  thermal_mass_Foster=[.001, .005, .05, .5] J/K  thermal_time_constant=[.001, .2] s  thermal_time_constant_Cauer=[.001, .1, .2] s  thermal_time_constant_Foster=[7e-05, .0007, .01, .08] s  thermal_mass_initial_temperatures=[25, 25] degC  thermal_mass_initial_temperatures_Cauer=[25, 25, 25] degC  junction_thermal_mass=0.01 J/K  Tvec_initial_Foster=[25, 25, 25, 25] degC  RthDiode=[.03, .2] K/W  RthCauerDiode=[.03, .1, .2] K/W  RthFosterDiode=[.03, .2] K/W  thermalMassDiode=[3, 25] J/K  thermalMassCauerDiode=[3, 10, 25] J/K  thermalMassFosterDiode=[33, 50] J/K  thermalTauDiode=[.1, 5] s  thermalTauCauerDiode=[.1, 1, 5] s  thermalTauFosterDiode=[1, 10] s  thermalMassInitTempDiode=[25, 25] degC  thermalMassInitTempCauerDiode=[25, 25, 25] degC  junctionthermalMassDiode=0.1 J/K  TVecInitialFosterDiode=[25, 25, 25, 25] degC  no_thermal_network=0  IGBT_junction_temperature_specify=off  IGBT_junction_temperature_priority=None  IGBT_junction_temperature=25 degC  IGBT_junction_temperature_nominal_specify=off  IGBT_junction_temperature_nominal_value=1  IGBT_junction_temperature_nominal_unit=degC  diode_junction_temperature_specify=off  diode_junction_temperature_priority=None  diode_junction_temperature=25 degC  diode_junction_temperature_nominal_specify=off  diode_junction_temperature_nominal_value=1  diode_junction_temperature_nominal_unit=degC  Qj_specify=off  Qj_priority=None  Qj=0 W  Qj_nominal_specify=off  Qj_nominal_value=1  Qj_nominal_unit=W  accumulatedSwitchingLosses_specify=off  accumulatedSwitchingLosses_priority=None  accumulatedSwitchingLosses=0 J
  Tb : ee_lib/Semiconductors & Converters/IGBT (Ideal, Switching)  port_option=ee.enum.controlport.ps  Vf=0.8 V  Ron=0.001 Ohm  Goff=1e-5 1/Ohm  Vth=0.5 V  diode_param=1  diode_Vf=0.8 V  diode_Ron=0.001 Ohm  diode_Goff=1e-5 1/Ohm  diode_C=5e-8 F  diode_iRM=-235 A  diode_iF=300 A  diode_idot=-50 A/us  diode_trr_param=1  diode_trr_factor=3  diode_trr=15 us  diode_Qrr=1.5e+3 s*uA  ice_specify=off  ice_priority=None  ice=0 A  ice_nominal_specify=off  ice_nominal_value=1  ice_nominal_unit=A  vce_specify=off  vce_priority=None  vce=0 V  vce_nominal_specify=off  vce_nominal_value=1  vce_nominal_unit=V  vge_specify=off  vge_priority=None  vge=0 V  vge_nominal_specify=off  vge_nominal_value=1  vge_nominal_unit=V  thermal_loss_option=ee.enum.converters.thermalLossOption.constantvalues  Von_data=[0, .1, .6, .8, 1, 1.3, 1.6, 2, 2.4; 0, .1, .7, 1, 1.2, 1.5, 1.9, 2.4, 2.8] V  Tj=[298.15, 398.15] K  Iout_data=[0, .1, 1, 5, 10, 20, 40, 70, 100] A  tabulateWithVce=false  Eon_data=[0, .0024, .024, .12, .2, .48, 1.04, 2.16, 3.24; 0, .003, .03, .15, .25, .6, 1.3, 2.7, 4.05] * 1e-3 J  Eoff_data=[0, .0007, .0066, .033, .066, .17, .33, .83, 1.5; 0, .001, .01, .05, .1, .25, .5, 1.2, 2.2] * 1e-3 J  Eon_data_3D=[zeros(2, 9, 3)] J  Eoff_data_3D=[zeros(2, 9, 3)] J  Tj_loss=[298.15, 398.15] K  Iout_data_loss=[0, .1, 1, 5, 10, 20, 40, 70, 100] A  Vce_loss=[0, 150, 300] V  Eon_scalar=22.86e-3 J  Eoff_scalar=17.14e-3 J  Voff=300 V  Iout_scalar=600 A  useCurrentFromPreviousCycle=false  useVoltageFromPreviousCycle=false  diodeModelType=ee.enum.converters.diodeModelType.pwl  diodeTableType=ee.enum.diode.tableType.IfMat  diode_ReverseIVType=ee.enum.diode.diodeReverseIV.constant  diode_IfMat=[.07, .12, .19, 1.75, 4.24, 7.32, 11.2; .16, .3, .72, 2.14, 4.02, 6.35, 9.12] A  diode_VfMat=[.9, 1.15, 1.25, 1.5, 1.75, 2.17, 2.6, 2.85; .58, .68, .75, 1.1, 1.38, 1.77, 2.27, 2.7] V  diode_TjVec=[25, 125] degC  diode_VfVec=[.5, .7, .9, 1.3, 1.7, 2.1, 2.5] V  diode_IfVec=[.1, .2, .5, 1, 2, 4, 7, 10] A  diode_IrMat=[1e-06, 2e-06, 5e-06, 1e-05, 2.5e-05, 5e-05, .0001; 2e-06, 5e-06, 1e-05, 4e-05, 8e-05, .0002, .0005] A  diode_VrMat=[10, 100, 200, 250, 300, 325, 350; 10, 70, 160, 220, 270, 300, 320] V  diode_VrVec=[10, 20, 40, 50, 70, 80, 100] V  diode_IrVec=[1e-06, 2e-06, 5e-06, 1e-05, 2e-05, 5e-05, .0001] A  diode_Vr=-600 V  diode_Ls=150 nH  diode_Erec=0.03 J  diode_rec_loss_model=ee.enum.diode.reverseRecoveryModel.fixed  diode_ErecVal=0 J  diode_scaleWithIandV=true  diode_ErecMat=zeros(2, 3) J  diodeErecMat3D=zeros(2, 3, 2) J  diode_TjrecVec=[298.15, 398.15] K  diode_IfrecVec=[.1, 1, 10] A  diodeVrecVec=[0, 100] V  diode_IrecVal=10 A  diode_VrecVal=10 V  diode_tFilter=1 / 1000 / 100 s  separateThermalPortForDiode=false  thermal_network_parameterization=ee.enum.thermalNetworkTopology.external  Rth=[.08, .5] K/W  Rth_Cauer=[.08, .1, .5] K/W  Rth_Foster=[.08, .14, .22, .16] K/W  thermal_mass_parameterization=ee.enum.thermalNetwork.timeconstant  thermal_mass=[.01, .5] J/K  thermal_mass_Cauer=[.01, .1, .5] J/K  thermal_mass_Foster=[.001, .005, .05, .5] J/K  thermal_time_constant=[.001, .2] s  thermal_time_constant_Cauer=[.001, .1, .2] s  thermal_time_constant_Foster=[7e-05, .0007, .01, .08] s  thermal_mass_initial_temperatures=[25, 25] degC  thermal_mass_initial_temperatures_Cauer=[25, 25, 25] degC  junction_thermal_mass=0.01 J/K  Tvec_initial_Foster=[25, 25, 25, 25] degC  RthDiode=[.03, .2] K/W  RthCauerDiode=[.03, .1, .2] K/W  RthFosterDiode=[.03, .2] K/W  thermalMassDiode=[3, 25] J/K  thermalMassCauerDiode=[3, 10, 25] J/K  thermalMassFosterDiode=[33, 50] J/K  thermalTauDiode=[.1, 5] s  thermalTauCauerDiode=[.1, 1, 5] s  thermalTauFosterDiode=[1, 10] s  thermalMassInitTempDiode=[25, 25] degC  thermalMassInitTempCauerDiode=[25, 25, 25] degC  junctionthermalMassDiode=0.1 J/K  TVecInitialFosterDiode=[25, 25, 25, 25] degC  no_thermal_network=0  IGBT_junction_temperature_specify=off  IGBT_junction_temperature_priority=None  IGBT_junction_temperature=25 degC  IGBT_junction_temperature_nominal_specify=off  IGBT_junction_temperature_nominal_value=1  IGBT_junction_temperature_nominal_unit=degC  diode_junction_temperature_specify=off  diode_junction_temperature_priority=None  diode_junction_temperature=25 degC  diode_junction_temperature_nominal_specify=off  diode_junction_temperature_nominal_value=1  diode_junction_temperature_nominal_unit=degC  Qj_specify=off  Qj_priority=None  Qj=0 W  Qj_nominal_specify=off  Qj_nominal_value=1  Qj_nominal_unit=W  accumulatedSwitchingLosses_specify=off  accumulatedSwitchingLosses_priority=None  accumulatedSwitchingLosses=0 J
  Tc : ee_lib/Semiconductors & Converters/IGBT (Ideal, Switching)  port_option=ee.enum.controlport.ps  Vf=0.8 V  Ron=0.001 Ohm  Goff=1e-5 1/Ohm  Vth=0.5 V  diode_param=1  diode_Vf=0.8 V  diode_Ron=0.001 Ohm  diode_Goff=1e-5 1/Ohm  diode_C=5e-8 F  diode_iRM=-235 A  diode_iF=300 A  diode_idot=-50 A/us  diode_trr_param=1  diode_trr_factor=3  diode_trr=15 us  diode_Qrr=1.5e+3 s*uA  ice_specify=off  ice_priority=None  ice=0 A  ice_nominal_specify=off  ice_nominal_value=1  ice_nominal_unit=A  vce_specify=off  vce_priority=None  vce=0 V  vce_nominal_specify=off  vce_nominal_value=1  vce_nominal_unit=V  vge_specify=off  vge_priority=None  vge=0 V  vge_nominal_specify=off  vge_nominal_value=1  vge_nominal_unit=V  thermal_loss_option=ee.enum.converters.thermalLossOption.constantvalues  Von_data=[0, .1, .6, .8, 1, 1.3, 1.6, 2, 2.4; 0, .1, .7, 1, 1.2, 1.5, 1.9, 2.4, 2.8] V  Tj=[298.15, 398.15] K  Iout_data=[0, .1, 1, 5, 10, 20, 40, 70, 100] A  tabulateWithVce=false  Eon_data=[0, .0024, .024, .12, .2, .48, 1.04, 2.16, 3.24; 0, .003, .03, .15, .25, .6, 1.3, 2.7, 4.05] * 1e-3 J  Eoff_data=[0, .0007, .0066, .033, .066, .17, .33, .83, 1.5; 0, .001, .01, .05, .1, .25, .5, 1.2, 2.2] * 1e-3 J  Eon_data_3D=[zeros(2, 9, 3)] J  Eoff_data_3D=[zeros(2, 9, 3)] J  Tj_loss=[298.15, 398.15] K  Iout_data_loss=[0, .1, 1, 5, 10, 20, 40, 70, 100] A  Vce_loss=[0, 150, 300] V  Eon_scalar=22.86e-3 J  Eoff_scalar=17.14e-3 J  Voff=300 V  Iout_scalar=600 A  useCurrentFromPreviousCycle=false  useVoltageFromPreviousCycle=false  diodeModelType=ee.enum.converters.diodeModelType.pwl  diodeTableType=ee.enum.diode.tableType.IfMat  diode_ReverseIVType=ee.enum.diode.diodeReverseIV.constant  diode_IfMat=[.07, .12, .19, 1.75, 4.24, 7.32, 11.2; .16, .3, .72, 2.14, 4.02, 6.35, 9.12] A  diode_VfMat=[.9, 1.15, 1.25, 1.5, 1.75, 2.17, 2.6, 2.85; .58, .68, .75, 1.1, 1.38, 1.77, 2.27, 2.7] V  diode_TjVec=[25, 125] degC  diode_VfVec=[.5, .7, .9, 1.3, 1.7, 2.1, 2.5] V  diode_IfVec=[.1, .2, .5, 1, 2, 4, 7, 10] A  diode_IrMat=[1e-06, 2e-06, 5e-06, 1e-05, 2.5e-05, 5e-05, .0001; 2e-06, 5e-06, 1e-05, 4e-05, 8e-05, .0002, .0005] A  diode_VrMat=[10, 100, 200, 250, 300, 325, 350; 10, 70, 160, 220, 270, 300, 320] V  diode_VrVec=[10, 20, 40, 50, 70, 80, 100] V  diode_IrVec=[1e-06, 2e-06, 5e-06, 1e-05, 2e-05, 5e-05, .0001] A  diode_Vr=-600 V  diode_Ls=150 nH  diode_Erec=0.03 J  diode_rec_loss_model=ee.enum.diode.reverseRecoveryModel.fixed  diode_ErecVal=0 J  diode_scaleWithIandV=true  diode_ErecMat=zeros(2, 3) J  diodeErecMat3D=zeros(2, 3, 2) J  diode_TjrecVec=[298.15, 398.15] K  diode_IfrecVec=[.1, 1, 10] A  diodeVrecVec=[0, 100] V  diode_IrecVal=10 A  diode_VrecVal=10 V  diode_tFilter=1 / 1000 / 100 s  separateThermalPortForDiode=false  thermal_network_parameterization=ee.enum.thermalNetworkTopology.external  Rth=[.08, .5] K/W  Rth_Cauer=[.08, .1, .5] K/W  Rth_Foster=[.08, .14, .22, .16] K/W  thermal_mass_parameterization=ee.enum.thermalNetwork.timeconstant  thermal_mass=[.01, .5] J/K  thermal_mass_Cauer=[.01, .1, .5] J/K  thermal_mass_Foster=[.001, .005, .05, .5] J/K  thermal_time_constant=[.001, .2] s  thermal_time_constant_Cauer=[.001, .1, .2] s  thermal_time_constant_Foster=[7e-05, .0007, .01, .08] s  thermal_mass_initial_temperatures=[25, 25] degC  thermal_mass_initial_temperatures_Cauer=[25, 25, 25] degC  junction_thermal_mass=0.01 J/K  Tvec_initial_Foster=[25, 25, 25, 25] degC  RthDiode=[.03, .2] K/W  RthCauerDiode=[.03, .1, .2] K/W  RthFosterDiode=[.03, .2] K/W  thermalMassDiode=[3, 25] J/K  thermalMassCauerDiode=[3, 10, 25] J/K  thermalMassFosterDiode=[33, 50] J/K  thermalTauDiode=[.1, 5] s  thermalTauCauerDiode=[.1, 1, 5] s  thermalTauFosterDiode=[1, 10] s  thermalMassInitTempDiode=[25, 25] degC  thermalMassInitTempCauerDiode=[25, 25, 25] degC  junctionthermalMassDiode=0.1 J/K  TVecInitialFosterDiode=[25, 25, 25, 25] degC  no_thermal_network=0  IGBT_junction_temperature_specify=off  IGBT_junction_temperature_priority=None  IGBT_junction_temperature=25 degC  IGBT_junction_temperature_nominal_specify=off  IGBT_junction_temperature_nominal_value=1  IGBT_junction_temperature_nominal_unit=degC  diode_junction_temperature_specify=off  diode_junction_temperature_priority=None  diode_junction_temperature=25 degC  diode_junction_temperature_nominal_specify=off  diode_junction_temperature_nominal_value=1  diode_junction_temperature_nominal_unit=degC  Qj_specify=off  Qj_priority=None  Qj=0 W  Qj_nominal_specify=off  Qj_nominal_value=1  Qj_nominal_unit=W  accumulatedSwitchingLosses_specify=off  accumulatedSwitchingLosses_priority=None  accumulatedSwitchingLosses=0 J
  + : PMIOPort  Side=Right
  0 : PMIOPort  Port=2  Side=Right
  - : PMIOPort  Port=3  Side=Right
  ~ : PMIOPort  Port=4  Side=Left
  wires:
  Demux/1 -> Simulink-PS Converter/1
  G/1 -> Demux/1
  Demux/2 -> Simulink-PS Converter1/1
  Demux/3 -> Simulink-PS Converter2/1
  connections:
  Dsc4/RConn1 -- 0/RConn1 -- Dsc3/LConn1 -- Dsb3/LConn1 -- Dsa3/LConn1 -- Dsa4/RConn1 -- Dsb4/RConn1
  Db2/LConn1 -- -/RConn1 -- Dc2/LConn1 -- Da2/LConn1
  Dc1/RConn1 -- +/RConn1 -- Da1/RConn1 -- Db1/RConn1
  Dsb1/LConn1 -- Dsb2/RConn1 -- Phase Splitter/RConn2
  Simulink-PS Converter1/RConn1 -- Tb/LConn1
  Dsb2/LConn1 -- Dsb4/LConn1 -- Tb/RConn2 -- Db2/RConn1
  Simulink-PS Converter2/RConn1 -- Tc/LConn1
  Dsb3/RConn1 -- Dsb1/RConn1 -- Db1/LConn1 -- Tb/RConn1
  Dsc2/LConn1 -- Dsc4/LConn1 -- Tc/RConn2 -- Dc2/RConn1
  Simulink-PS Converter/RConn1 -- Ta/LConn1
  Dsa1/LConn1 -- Phase Splitter/RConn1 -- Dsa2/RConn1
  Dsa1/RConn1 -- Dsa3/RConn1 -- Da1/LConn1 -- Ta/RConn1
  Dsc1/LConn1 -- Dsc2/RConn1 -- Phase Splitter/RConn3
  Dsc1/RConn1 -- Dsc3/RConn1 -- Dc1/LConn1 -- Tc/RConn1
  Ta/RConn2 -- Dsa2/LConn1 -- Da2/RConn1 -- Dsa4/LConn1
  ~/RConn1 -- Phase Splitter/LConn1
